simulink model "prosjektoppgave_4_"  (R2026a)
settings: Solver=VariableStepAuto  StopTime=100  MaxStep=0.01
values from neighbouring files (symbols this model uses):
  A = pi*(1/2)^2    (= 0.785398163397)    [Ferdig tunet.m]
  At = pi*(0.075)^2    (= 0.0176714586764)    [Ferdig tunet.m]
  Atut = At/2    (= 0.00883572933822)    [Ferdig tunet.m]
  hf = 0    [Ferdig tunet.m]
  href = 0.6    [Ferdig tunet.m]
  k = sqrt(2*9.81)*1000*Atut/2    [Ferdig tunet.m]
  Kd = 2    [Ferdig tunet.m]
  Kd4 = 2.1    [Ferdig tunet.m]
  Ki = 0.0025    [Ferdig tunet.m]
  Ki2 = 0.034    [Ferdig tunet.m]
  Kp = 8    [Ferdig tunet.m]
  Kp1 = 10    [Ferdig tunet.m]
  Kp2 = 0.39    [Ferdig tunet.m]
  Kp3 = 3    [Ferdig tunet.m]
  Kp4 = 30    [Ferdig tunet.m]
  L = 0.1    [Ferdig tunet.m]
  p = 1000    [Ferdig tunet.m]
undefined symbols (not defined in the file or in its folder): gammaverdi, h, h10, h20, omega_0, r, rt, zeta
libraries: vrlib x1
settings Model: Creator=User  LastModifiedBy=arnes

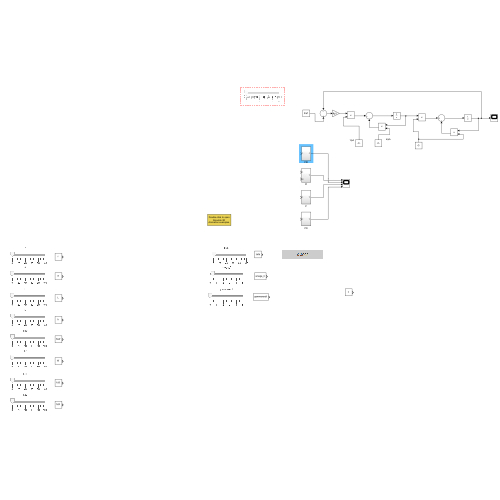
[thumbnail: Simulink's stored preview of the top-level diagram]
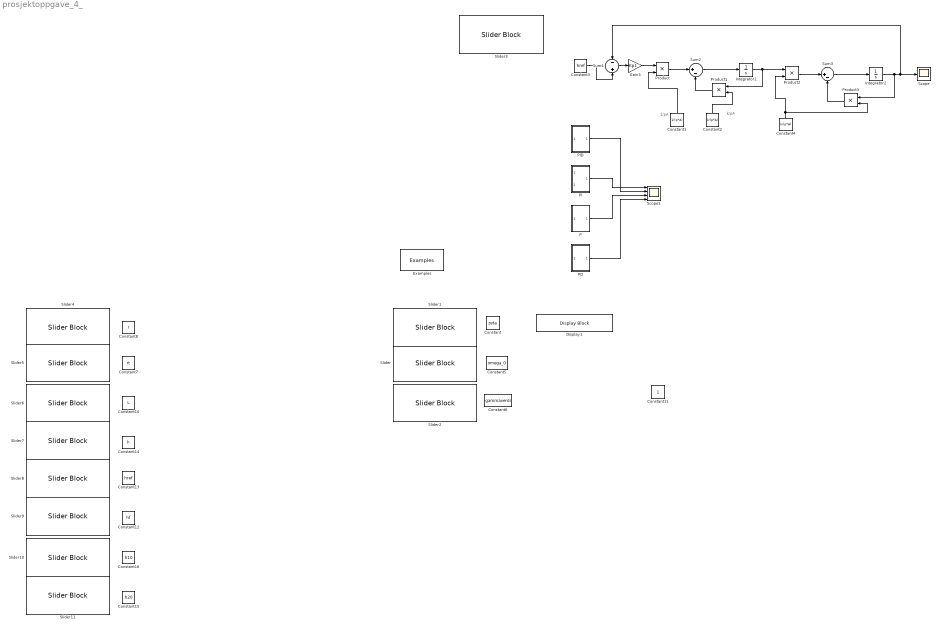
== system prosjektoppgave_4_ ==
  note: 1/pA
  note: k/pA
  Constant : Constant  Value=zeta
  Constant1 : Constant  Value=1/(p*A)
  Constant10 : Constant  Value=L
  Constant11 : Constant
  Constant12 : Constant  Value=hf
  Constant13 : Constant  Value=href
  Constant14 : Constant  Value=h
  Constant15 : Constant  Value=h20
  Constant16 : Constant  Value=h10
  Constant2 : Constant  Value=k/(p*A)
  Constant3 : Constant  Value=href
  Constant4 : Constant  Value=k/(p*A)
  Constant5 : Constant  Value=omega_0
  Constant6 : Constant  Value=gammaverdi
  Constant7 : Constant  Value=rt
  Constant8 : Constant  Value=r
  Display1 : DisplayBlock  LabelPosition=Hide  Transparency=1  GridColor=[0.502, 0.502, 0.502]
  Examples : vrlib/Examples
  Gain3 : Gain  Gain=Kp1
  Integrator1 : Integrator  InitialCondition=0.8
  Integrator2 : Integrator  InitialCondition=0.6
  P : Subsystem
  PD : Subsystem
  PI : Subsystem
  PID : Subsystem
  Product{,1..3} (4 alike) : Product
  Scope : Scope
      settings: ActiveDisplayYMinimum=-0.5025354614211307  ActiveDisplayYMaximum=0.76642979259143185  DataLoggingVariableName=ScopeData3  DataLoggingSaveFormat=Array
  Scope1 : Scope  NumInputPorts=4
      settings: ActiveDisplayYMinimum=0.58592431885345853  ActiveDisplayYMaximum=0.88083018468333463  DataLoggingVariableName=ScopeData4
  Slider : SliderBlock  ScaleMax=5
  Slider{1,4..11} (9 alike) : SliderBlock
  Slider2 : SliderBlock  ScaleMax=5
  Slider3 : SliderBlock  ScaleMax=5
  Sum2 : Sum  Inputs=|+-
  Sum3 : Sum  Inputs=|+-
  Sum4 : Sum  Inputs=-+
  wires:
  Gain3/1 -> Product/1
  Sum3/1 -> Integrator2/1
  Constant4/1 -> Product3/2, Product2/2
  Integrator1/1 -> Product2/1, Product1/1
  Constant1/1 -> Product/2
  Product3/1 -> Sum3/2
  Sum4/1 -> Gain3/1
  Constant3/1 -> Sum4/2
  Sum2/1 -> Integrator1/1
  Product/1 -> Sum2/1
  Constant2/1 -> Product1/2
  Product1/1 -> Sum2/2
  Product2/1 -> Sum3/1
  Integrator2/1 -> Sum4/1, Scope/1, Product3/1
  PID/1(Out1) -> Scope1/2
  PI/1(Out1) -> Scope1/1
  P/1(Out1) -> Scope1/3
  PD/1(Out1) -> Scope1/4

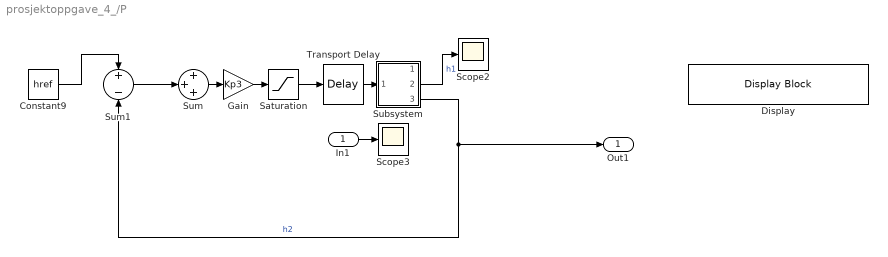
== system prosjektoppgave_4_/P ==
  In1 : Inport
  Constant9 : Constant  Value=href
  Display : DisplayBlock  LabelPosition=Hide  Transparency=1  GridColor=[0.502, 0.502, 0.502]
  Gain : Gain  Gain=Kp3
  Saturation : Saturate
  Scope2 : Scope
      settings: ActiveDisplayYMinimum=-1  ActiveDisplayYMaximum=1  DataLoggingVariableName=ScopeData2  DataLoggingSaveFormat=Array
  Scope3 : Scope
      settings: ActiveDisplayYMinimum=-0.49116355896890118  ActiveDisplayYMaximum=0.71407060545940459  DataLoggingSaveFormat=Array
  Subsystem : Subsystem
  Sum : Sum  Inputs=+++
  Sum1 : Sum  Inputs=+-
  Transport Delay : TransportDelay  DelayTime=(2*L)/(sqrt(2*9.81))
  Out1 : Outport
  wires:
  Constant9/1 -> Sum1/1
  Subsystem/3(Out2) -> Out1/1, Sum1/2  "h2"
  Subsystem/2(Out1) -> Scope2/1  "h1"
  Sum1/1 -> Sum/2
  Sum/1 -> Gain/1
  Transport Delay/1 -> Subsystem/1(In1)
  In1/1 -> Scope3/1
  Gain/1 -> Saturation/1
  Saturation/1 -> Transport Delay/1

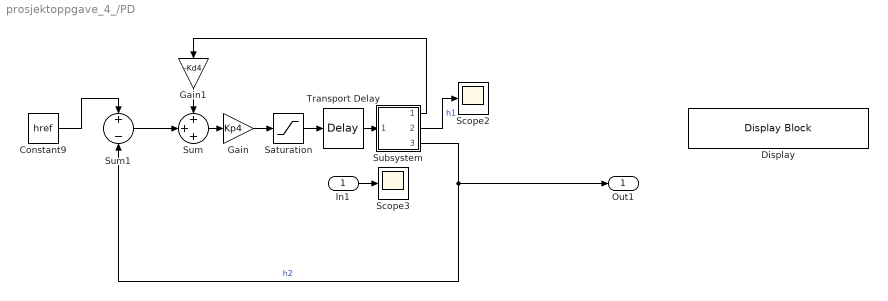
== system prosjektoppgave_4_/PD ==
  In1 : Inport
  Constant9 : Constant  Value=href
  Display : DisplayBlock  LabelPosition=Hide  Transparency=1  GridColor=[0.502, 0.502, 0.502]
  Gain : Gain  Gain=Kp4
  Gain1 : Gain  Gain=-Kd4
  Saturation : Saturate
  Scope2 : Scope
      settings: ActiveDisplayYMinimum=-1  ActiveDisplayYMaximum=1  DataLoggingVariableName=ScopeData2  DataLoggingSaveFormat=Array
  Scope3 : Scope
      settings: ActiveDisplayYMinimum=-0.49116355896890118  ActiveDisplayYMaximum=0.71407060545940459  DataLoggingSaveFormat=Array
  Subsystem : Subsystem
  Sum : Sum  Inputs=+++
  Sum1 : Sum  Inputs=+-
  Transport Delay : TransportDelay  DelayTime=(2*L)/(sqrt(2*9.81))
  Out1 : Outport
  wires:
  Constant9/1 -> Sum1/1
  Subsystem/3(Out2) -> Out1/1, Sum1/2  "h2"
  Subsystem/1(Out3) -> Gain1/1
  Subsystem/2(Out1) -> Scope2/1  "h1"
  Sum1/1 -> Sum/2
  Sum/1 -> Gain/1
  Gain1/1 -> Sum/1
  Transport Delay/1 -> Subsystem/1(In1)
  In1/1 -> Scope3/1
  Saturation/1 -> Transport Delay/1
  Gain/1 -> Saturation/1

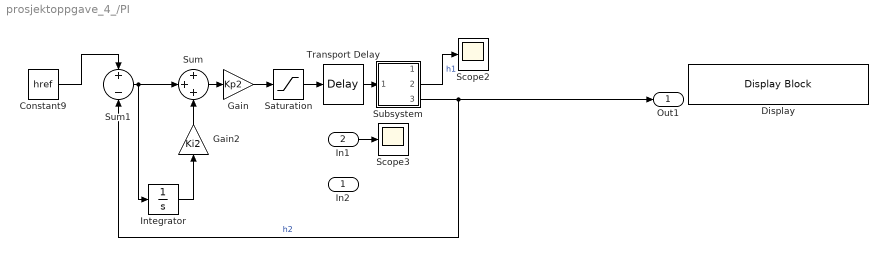
== system prosjektoppgave_4_/PI ==
  In2 : Inport
  In1 : Inport  Port=2
  Constant9 : Constant  Value=href
  Display : DisplayBlock  LabelPosition=Hide  Transparency=1  GridColor=[0.502, 0.502, 0.502]
  Gain : Gain  Gain=Kp2
  Gain2 : Gain  Gain=Ki2
  Integrator : Integrator
  Saturation : Saturate
  Scope2 : Scope
      settings: ActiveDisplayYMinimum=-1  ActiveDisplayYMaximum=1  DataLoggingVariableName=ScopeData2  DataLoggingSaveFormat=Array
  Scope3 : Scope
      settings: ActiveDisplayYMinimum=-0.49116355896890118  ActiveDisplayYMaximum=0.71407060545940459  DataLoggingSaveFormat=Array
  Subsystem : Subsystem
  Sum : Sum  Inputs=+++
  Sum1 : Sum  Inputs=+-
  Transport Delay : TransportDelay  DelayTime=(2*L)/(sqrt(2*9.81))
  Out1 : Outport
  wires:
  Constant9/1 -> Sum1/1
  Gain2/1 -> Sum/3
  Integrator/1 -> Gain2/1
  Subsystem/3(Out2) -> Out1/1, Sum1/2  "h2"
  Subsystem/2(Out1) -> Scope2/1  "h1"
  Sum1/1 -> Integrator/1, Sum/2
  Sum/1 -> Gain/1
  Transport Delay/1 -> Subsystem/1(In1)
  In1/1 -> Scope3/1
  Saturation/1 -> Transport Delay/1
  Gain/1 -> Saturation/1

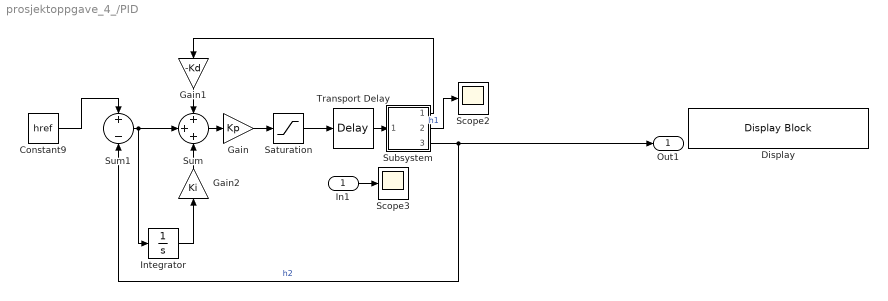
== system prosjektoppgave_4_/PID ==
  In1 : Inport
  Constant9 : Constant  Value=href
  Display : DisplayBlock  LabelPosition=Hide  Transparency=1  GridColor=[0.502, 0.502, 0.502]
  Gain : Gain  Gain=Kp
  Gain1 : Gain  Gain=-Kd
  Gain2 : Gain  Gain=Ki
  Integrator : Integrator
  Saturation : Saturate
  Scope2 : Scope
      settings: ActiveDisplayYMinimum=-1  ActiveDisplayYMaximum=1  DataLoggingVariableName=ScopeData2  DataLoggingSaveFormat=Array
  Scope3 : Scope
      settings: ActiveDisplayYMinimum=-0.49116355896890118  ActiveDisplayYMaximum=0.71407060545940459  DataLoggingSaveFormat=Array
  Subsystem : Subsystem
  Sum : Sum  Inputs=+++
  Sum1 : Sum  Inputs=+-
  Transport Delay : TransportDelay  DelayTime=(2*L)/(sqrt(2*9.81))
  Out1 : Outport
  wires:
  Constant9/1 -> Sum1/1
  Gain2/1 -> Sum/3
  Integrator/1 -> Gain2/1
  Subsystem/3(Out2) -> Out1/1, Sum1/2  "h2"
  Subsystem/1(Out3) -> Gain1/1
  Subsystem/2(Out1) -> Scope2/1  "h1"
  Sum1/1 -> Integrator/1, Sum/2
  Sum/1 -> Gain/1
  Gain1/1 -> Sum/1
  Transport Delay/1 -> Subsystem/1(In1)
  In1/1 -> Scope3/1
  Saturation/1 -> Transport Delay/1
  Gain/1 -> Saturation/1

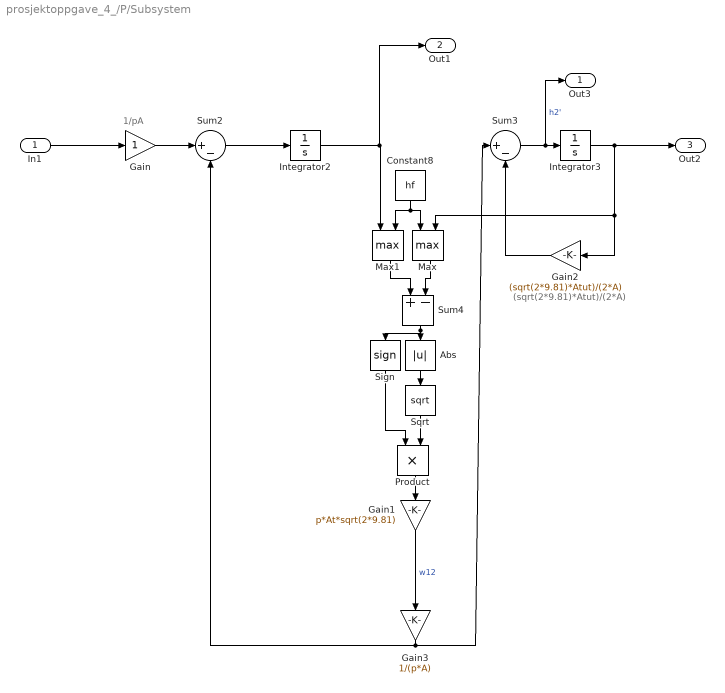
== system prosjektoppgave_4_/P/Subsystem ==
  note: (sqrt(2*9.81)*Atut)/(2*A)
  note: 1/pA
  In1 : Inport  OutMin=0
  Abs : Abs  SaturateOnIntegerOverflow=off
  Constant8 : Constant  Value=hf
  Gain : Gain
  Gain1 : Gain  Gain=p*At*sqrt(2*9.81)
  Gain2 : Gain  Gain=(sqrt(2*9.81)*Atut)/(2*A)
  Gain3 : Gain  Gain=1/(p*A)
  Integrator2 : Integrator  InitialCondition=0.8
  Integrator3 : Integrator  InitialCondition=0.6
  Max : MinMax  Function=max  Inputs=2
  Max1 : MinMax  Function=max  Inputs=2
  Product : Product
  Sign : Signum
  Sqrt : Sqrt
  Sum2 : Sum  Inputs=|+-
  Sum3 : Sum  Inputs=|+-
  Sum4 : Sum  Inputs=+-
  Out3 : Outport  VectorParamsAs1DForOutWhenUnconnected=off
  Out1 : Outport  Port=2
  Out2 : Outport  Port=3
  wires:
  Sum2/1 -> Integrator2/1
  Gain/1 -> Sum2/1
  Sum3/1 -> Out3/1, Integrator3/1  "h2'"
  Max1/1 -> Sum4/1
  Integrator2/1 -> Out1/1, Max1/1
  Constant8/1 -> Max1/2, Max/1
  Max/1 -> Sum4/2
  Integrator3/1 -> Out2/1, Gain2/1, Max/2
  Gain3/1 -> Sum3/1, Sum2/2
  Gain2/1 -> Sum3/2
  Abs/1 -> Sqrt/1
  Sum4/1 -> Sign/1, Abs/1
  Sign/1 -> Product/1
  Sqrt/1 -> Product/2
  Product/1 -> Gain1/1
  Gain1/1 -> Gain3/1  "w12"
  In1/1 -> Gain/1

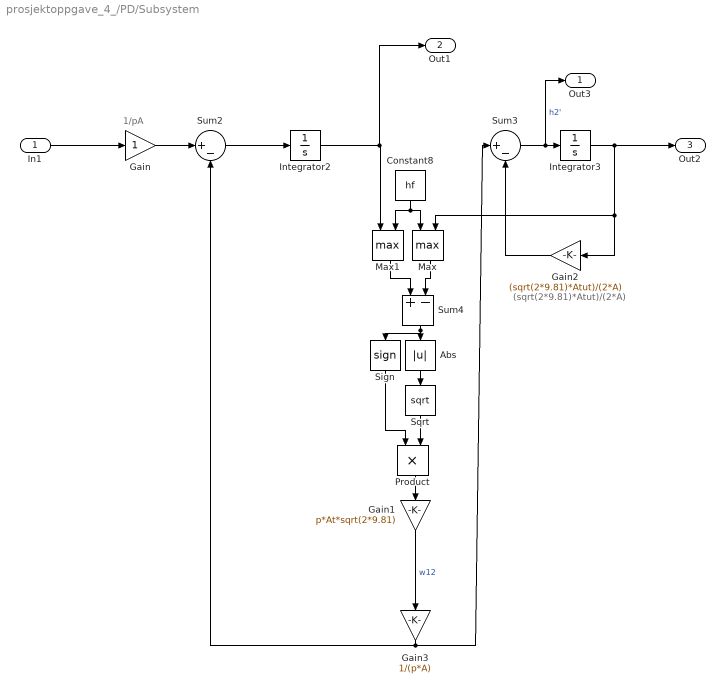
== system prosjektoppgave_4_/PD/Subsystem ==
  note: (sqrt(2*9.81)*Atut)/(2*A)
  note: 1/pA
  In1 : Inport  OutMin=0
  Abs : Abs  SaturateOnIntegerOverflow=off
  Constant8 : Constant  Value=hf
  Gain : Gain
  Gain1 : Gain  Gain=p*At*sqrt(2*9.81)
  Gain2 : Gain  Gain=(sqrt(2*9.81)*Atut)/(2*A)
  Gain3 : Gain  Gain=1/(p*A)
  Integrator2 : Integrator  InitialCondition=0.8
  Integrator3 : Integrator  InitialCondition=0.6
  Max : MinMax  Function=max  Inputs=2
  Max1 : MinMax  Function=max  Inputs=2
  Product : Product
  Sign : Signum
  Sqrt : Sqrt
  Sum2 : Sum  Inputs=|+-
  Sum3 : Sum  Inputs=|+-
  Sum4 : Sum  Inputs=+-
  Out3 : Outport  VectorParamsAs1DForOutWhenUnconnected=off
  Out1 : Outport  Port=2
  Out2 : Outport  Port=3
  wires:
  Sum2/1 -> Integrator2/1
  Gain/1 -> Sum2/1
  Sum3/1 -> Out3/1, Integrator3/1  "h2'"
  Max1/1 -> Sum4/1
  Integrator2/1 -> Out1/1, Max1/1
  Constant8/1 -> Max1/2, Max/1
  Max/1 -> Sum4/2
  Integrator3/1 -> Out2/1, Gain2/1, Max/2
  Gain3/1 -> Sum3/1, Sum2/2
  Gain2/1 -> Sum3/2
  Abs/1 -> Sqrt/1
  Sum4/1 -> Sign/1, Abs/1
  Sign/1 -> Product/1
  Sqrt/1 -> Product/2
  Product/1 -> Gain1/1
  Gain1/1 -> Gain3/1  "w12"
  In1/1 -> Gain/1

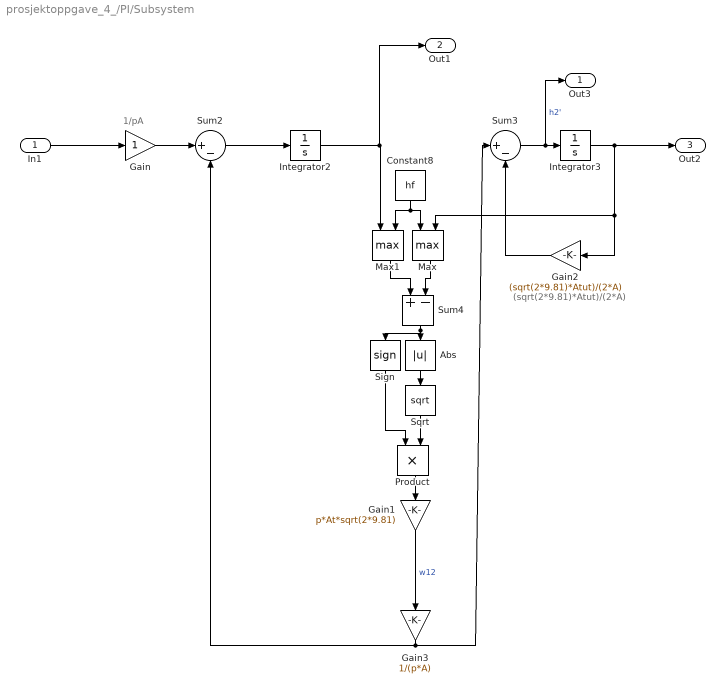
== system prosjektoppgave_4_/PI/Subsystem ==
  note: (sqrt(2*9.81)*Atut)/(2*A)
  note: 1/pA
  In1 : Inport  OutMin=0
  Abs : Abs  SaturateOnIntegerOverflow=off
  Constant8 : Constant  Value=hf
  Gain : Gain
  Gain1 : Gain  Gain=p*At*sqrt(2*9.81)
  Gain2 : Gain  Gain=(sqrt(2*9.81)*Atut)/(2*A)
  Gain3 : Gain  Gain=1/(p*A)
  Integrator2 : Integrator  InitialCondition=0.8
  Integrator3 : Integrator  InitialCondition=0.6
  Max : MinMax  Function=max  Inputs=2
  Max1 : MinMax  Function=max  Inputs=2
  Product : Product
  Sign : Signum
  Sqrt : Sqrt
  Sum2 : Sum  Inputs=|+-
  Sum3 : Sum  Inputs=|+-
  Sum4 : Sum  Inputs=+-
  Out3 : Outport  VectorParamsAs1DForOutWhenUnconnected=off
  Out1 : Outport  Port=2
  Out2 : Outport  Port=3
  wires:
  Sum2/1 -> Integrator2/1
  Gain/1 -> Sum2/1
  Sum3/1 -> Out3/1, Integrator3/1  "h2'"
  Max1/1 -> Sum4/1
  Integrator2/1 -> Out1/1, Max1/1
  Constant8/1 -> Max1/2, Max/1
  Max/1 -> Sum4/2
  Integrator3/1 -> Out2/1, Gain2/1, Max/2
  Gain3/1 -> Sum3/1, Sum2/2
  Gain2/1 -> Sum3/2
  Abs/1 -> Sqrt/1
  Sum4/1 -> Sign/1, Abs/1
  Sign/1 -> Product/1
  Sqrt/1 -> Product/2
  Product/1 -> Gain1/1
  Gain1/1 -> Gain3/1  "w12"
  In1/1 -> Gain/1

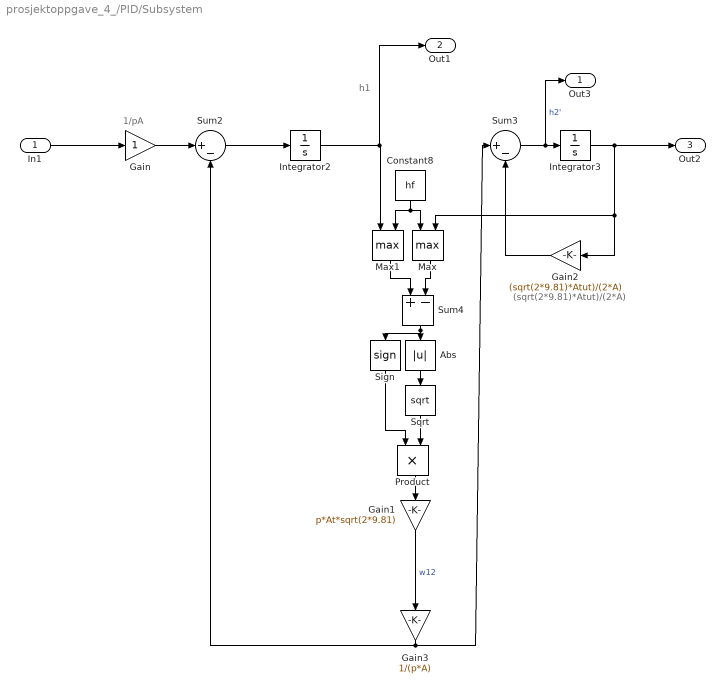
== system prosjektoppgave_4_/PID/Subsystem ==
  note: h1
  note: (sqrt(2*9.81)*Atut)/(2*A)
  note: 1/pA
  In1 : Inport  OutMin=0
  Abs : Abs  SaturateOnIntegerOverflow=off
  Constant8 : Constant  Value=hf
  Gain : Gain
  Gain1 : Gain  Gain=p*At*sqrt(2*9.81)
  Gain2 : Gain  Gain=(sqrt(2*9.81)*Atut)/(2*A)
  Gain3 : Gain  Gain=1/(p*A)
  Integrator2 : Integrator  InitialCondition=0.8
  Integrator3 : Integrator  InitialCondition=0.6
  Max : MinMax  Function=max  Inputs=2
  Max1 : MinMax  Function=max  Inputs=2
  Product : Product
  Sign : Signum
  Sqrt : Sqrt
  Sum2 : Sum  Inputs=|+-
  Sum3 : Sum  Inputs=|+-
  Sum4 : Sum  Inputs=+-
  Out3 : Outport  VectorParamsAs1DForOutWhenUnconnected=off
  Out1 : Outport  Port=2
  Out2 : Outport  Port=3
  wires:
  Sum2/1 -> Integrator2/1
  Gain/1 -> Sum2/1
  Sum3/1 -> Out3/1, Integrator3/1  "h2'"
  Max1/1 -> Sum4/1
  Integrator2/1 -> Out1/1, Max1/1
  Constant8/1 -> Max1/2, Max/1
  Max/1 -> Sum4/2
  Integrator3/1 -> Out2/1, Gain2/1, Max/2
  Gain3/1 -> Sum3/1, Sum2/2
  Gain2/1 -> Sum3/2
  Abs/1 -> Sqrt/1
  Sum4/1 -> Sign/1, Abs/1
  Sign/1 -> Product/1
  Sqrt/1 -> Product/2
  Product/1 -> Gain1/1
  Gain1/1 -> Gain3/1  "w12"
  In1/1 -> Gain/1
